simulink model "SpectatorFollowingVhcl"  (R2020a)
settings: Solver=FixedStepAuto  StartTime=0.0  StopTime=inf  FixedStep=0.1  RelTol=1e-3
libraries: Carla4SL x7
settings Model: Creator=IMM9  LastModifiedBy=IMM9

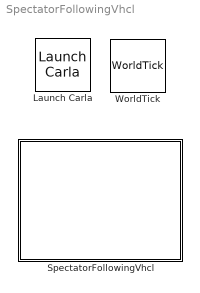
== system SpectatorFollowingVhcl ==
  Launch Carla : Carla4SL/Carla Environment/Launch Carla  Port=2000  Timeout=20  CarlaPath=[]  Width=600  Height=340  SimulationMode=Synchronous  Quality=Epic  Map=Town01  Weather=ClearNoon  NPCs=0
      settings: SourceProductName=Carla for Simulink
  SpectatorFollowingVhcl : Subsystem
  WorldTick : Carla4SL/Carla Environment/WorldTick
      settings: SourceProductName=Carla for Simulink

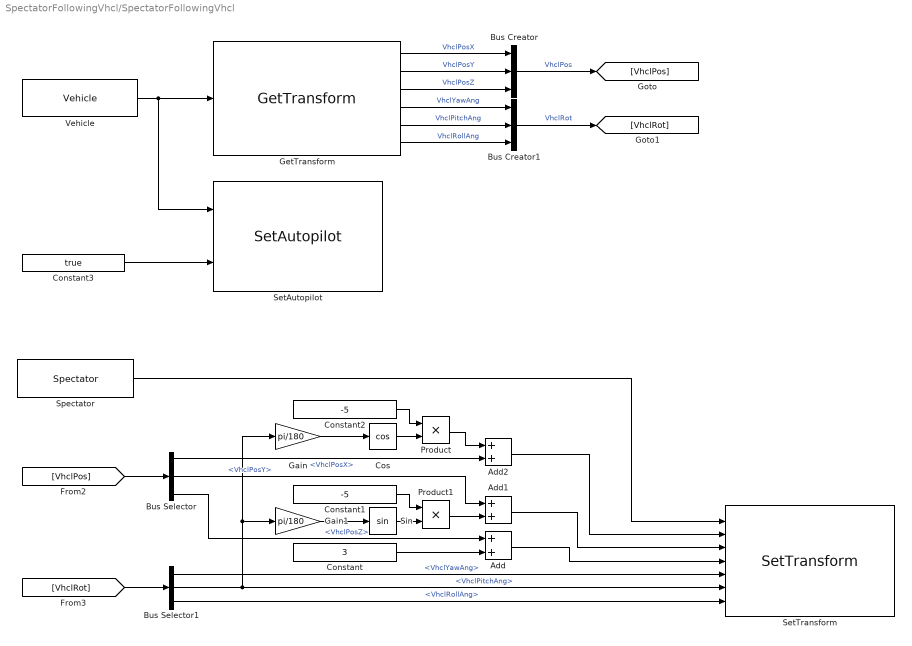
== system SpectatorFollowingVhcl/SpectatorFollowingVhcl ==
  Add : Sum
  Add1 : Sum
  Add2 : Sum
  Bus Creator : BusCreator  Inputs=3
  Bus Creator1 : BusCreator  Inputs=3
  Bus Selector : BusSelector  OutputSignals=VhclPosX,VhclPosY,VhclPosZ
  Bus Selector1 : BusSelector  OutputSignals=VhclYawAng,VhclPitchAng,VhclRollAng
  Constant : Constant  Value=3  SampleTime=-1
  Constant1 : Constant  Value=-5  SampleTime=-1
  Constant2 : Constant  Value=-5  SampleTime=-1
  Constant3 : Constant  Value=true  OutDataTypeStr=boolean  SampleTime=-1
  Cos : Trigonometry  Operator=cos
  Gain : Gain  Gain=pi/180
  Gain1 : Gain  Gain=pi/180
  GetTransform : Carla4SL/Getters/GetTransform
      settings: SourceProductName=Carla for Simulink
  Product : Product
  Product1 : Product
  SetAutopilot : Carla4SL/Setters/SetAutopilot
      settings: SourceProductName=Carla for Simulink
  SetTransform : Carla4SL/Setters/SetTransform
      settings: SourceProductName=Carla for Simulink
  Sin : Trigonometry
  Spectator : Carla4SL/Actors/Spectator
      settings: SourceProductName=Carla for Simulink
  Vehicle : Carla4SL/Actors/Vehicle
      settings: SourceProductName=Carla for Simulink
  wires:
  GetTransform/3 -> Bus Creator/3  "VhclPosZ"
  GetTransform/2 -> Bus Creator/2  "VhclPosY"
  GetTransform/1 -> Bus Creator/1  "VhclPosX"
  GetTransform/5 -> Bus Creator1/2  "VhclPitchAng"
  GetTransform/6 -> Bus Creator1/3  "VhclRollAng"
  GetTransform/4 -> Bus Creator1/1  "VhclYawAng"
  Vehicle/1 -> SetAutopilot/1, GetTransform/1
  Bus Creator/1 -> [VhclPos]  "VhclPos"
  Bus Creator1/1 -> [VhclRot]  "VhclRot"
  [VhclPos] -> Bus Selector/1
  [VhclRot] -> Bus Selector1/1
  Bus Selector1/1 -> SetTransform/5  "<VhclYawAng>"
  Bus Selector/3 -> Add/1  "<VhclPosZ>"
  Constant/1 -> Add/2
  Sin/1 -> Product1/2
  Constant1/1 -> Product1/1
  Product1/1 -> Add1/2
  Cos/1 -> Product/2
  Constant2/1 -> Product/1
  Spectator/1 -> SetTransform/1
  Bus Selector/1 -> Add2/2  "<VhclPosX>"
  Product/1 -> Add2/1
  Bus Selector/2 -> Add1/1  "<VhclPosY>"
  Gain/1 -> Cos/1
  Gain1/1 -> Sin/1
  Constant3/1 -> SetAutopilot/2
  Bus Selector1/3 -> SetTransform/7  "<VhclRollAng>"
  Bus Selector1/2 -> Gain/1, Gain1/1, SetTransform/6  "<VhclPitchAng>"
  Add/1 -> SetTransform/4
  Add1/1 -> SetTransform/3
  Add2/1 -> SetTransform/2
